simulink model "NBMS_App"  (R2026b)
settings: Solver=FixedStepDiscrete  StopTime=25  FixedStep=0.1
undefined symbols (not defined in the file): BMS_HVMosfet_STS_E, BMS_MODE_E, BMS_NM_Msg_E, Charger_Mode_Req_E
settings Model: ModifiedByFormat=Hari  Creator=hp  LastModifiedBy=Hari
settings OptimizationCC: DefaultParameterBehavior=Inlined  DifferentSizesBufferReuse=on  EfficientTunableParamExpr=on  EnhancedBackFolding=on  OptimizationCustomize=off  OptimizeBlockOrder=speed  PassReuseOutputArgsAs=Individual arguments  RemoveInternalMemoryZeroInit=on  RemoveRootLevelIOMemoryZeroInit=on
settings DebuggingCC: ParameterTunabilityLossMsg=error
settings SFSimCC: MATLABDynamicMemAlloc=off
settings RTWCC: Description=Embedded Coder  GenCodeOnly=on  PackageGeneratedCodeAndArtifacts=on  SystemTargetFile=ert.tlc  TemplateMakefile=ert_default_tmf
settings CodeAppCC: ForceParamTrailComments=on  IgnoreCustomStorageClasses=off  InsertBlockDesc=on  OperatorAnnotations=on  SFDataObjDesc=on  SimulinkDataObjDesc=on
settings ERTTargetCC: DynamicArrayContainerType=coder::array  GenerateSampleERTMain=on
settings ConfigComp: DVDefectChecker=on  DVDetectOutOfBounds=on  DVHarnessSource=Signal Editor  DVModelReferenceHarness=on  DVTestSuiteOptimization=Auto

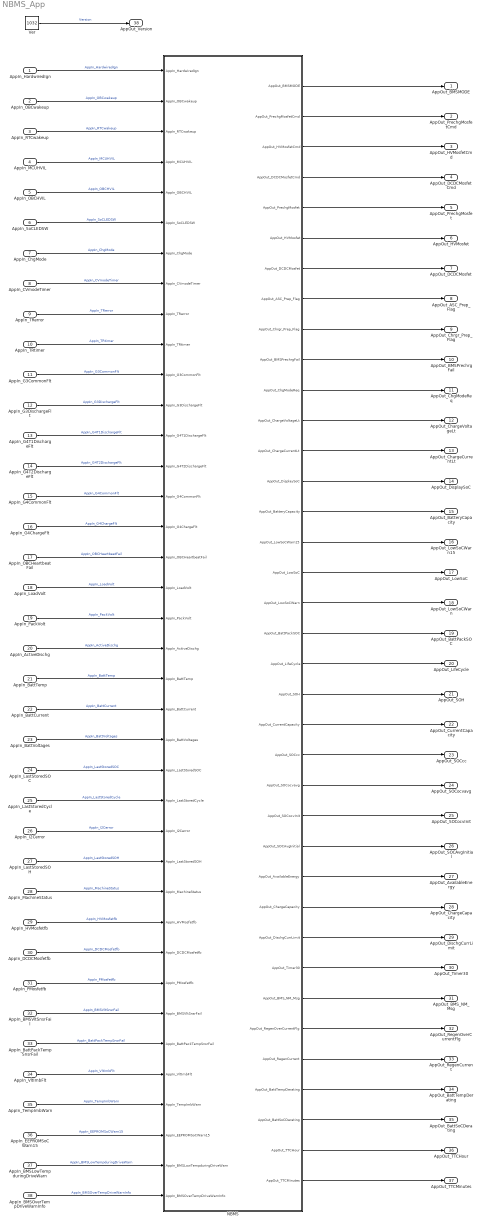
== system NBMS_App ==
  AppIn_HardwiredIgn : Inport  OutMin=0  OutMax=1  OutDataTypeStr=boolean
  AppIn_OBCwakeup : Inport  Port=2  OutDataTypeStr=Enum: OBC_E
  AppIn_RTCwakeup : Inport  Port=3  OutMin=0  OutMax=1  OutDataTypeStr=boolean
  AppIn_MCUHVIL : Inport  Port=4  OutMin=0  OutMax=1  OutDataTypeStr=boolean
  AppIn_OBCHVIL : Inport  Port=5  OutMin=0  OutMax=1  OutDataTypeStr=boolean
  AppIn_SoCLEDSW : Inport  Port=6  OutMin=0  OutMax=1  OutDataTypeStr=boolean
  AppIn_ChgMode : Inport  Port=7  OutDataTypeStr=Enum: Charger_Mode_E
  AppIn_CVmodeTimer : Inport  Port=8  OutDataTypeStr=Enum: CV_Mode_Timer_E
  AppIn_TRerror : Inport  Port=9  OutMin=0  OutMax=1  OutDataTypeStr=boolean
  AppIn_TRtimer : Inport  Port=10  OutMin=0  OutMax=1  OutDataTypeStr=boolean
  AppIn_G3CommonFlt : Inport  Port=11  OutMin=0  OutMax=1  OutDataTypeStr=boolean
  AppIn_G3DischargeFlt : Inport  Port=12  OutMin=0  OutMax=1  OutDataTypeStr=boolean
  AppIn_G4T1DischargeFlt : Inport  Port=13  OutMin=0  OutMax=1  OutDataTypeStr=boolean
  AppIn_G4T2DischargeFlt : Inport  Port=14  OutMin=0  OutMax=1  OutDataTypeStr=boolean
  AppIn_G4CommonFlt : Inport  Port=15  OutMin=0  OutMax=1  OutDataTypeStr=boolean
  AppIn_G4ChargeFlt : Inport  Port=16  OutMin=0  OutMax=1  OutDataTypeStr=boolean
  AppIn_OBCHeartbeatFail : Inport  Port=17  OutMin=0  OutMax=1  OutDataTypeStr=boolean
  AppIn_LoadVolt : Inport  Port=18  OutDataTypeStr=double
  AppIn_PackVolt : Inport  Port=19  OutDataTypeStr=double
  AppIn_ActiveDischg : Inport  Port=20  OutDataTypeStr=Enum: Active_DisChrg_E
  AppIn_BattTemp : Inport  Port=21  OutDataTypeStr=double  PortDimensions=[6,1]
  AppIn_BattCurrent : Inport  Port=22  OutDataTypeStr=double
  AppIn_BattVoltages : Inport  Port=23  OutDataTypeStr=double  PortDimensions=[20,1]
  AppIn_LastStoredSOC : Inport  Port=24  OutMin=0  OutMax=100  OutDataTypeStr=double
  AppIn_LastStoredCycle : Inport  Port=25  OutDataTypeStr=double
  AppIn_I2Cerror : Inport  Port=26  OutMin=0  OutMax=1  OutDataTypeStr=boolean
  AppIn_LastStoredSOH : Inport  Port=27  OutMin=0  OutMax=100  OutDataTypeStr=double
  AppIn_MachineStatus : Inport  Port=28  OutDataTypeStr=Enum: VDU_MACHINE_STS_E
  AppIn_HVMosfetfb : Inport  Port=29  OutMin=0  OutMax=1  OutDataTypeStr=boolean
  AppIn_DCDCMosfetfb : Inport  Port=30  OutMin=0  OutMax=1  OutDataTypeStr=boolean
  AppIn_PMosfetfb : Inport  Port=31  OutMin=0  OutMax=1  OutDataTypeStr=boolean
  AppIn_BMSVltSnsrFail : Inport  Port=32  OutMin=0  OutMax=1  OutDataTypeStr=boolean
  AppIn_BattPackTempSnsrFail : Inport  Port=33  OutMin=0  OutMax=1  OutDataTypeStr=boolean
  AppIn_VltImbFlt : Inport  Port=34  OutMin=0  OutMax=1  OutDataTypeStr=boolean
  AppIn_TempImbWarn : Inport  Port=35  OutMin=0  OutMax=1  OutDataTypeStr=boolean
  AppIn_EEPROMSoCWarn15 : Inport  Port=36  OutDataTypeStr=boolean
  AppIn_BMSLowTempduringDriveWarn : Inport  Port=37  OutDataTypeStr=boolean
  AppIn_BMSOverTempDriveWarnInfo : Inport  Port=38  OutDataTypeStr=boolean
  NBMS : Subsystem
  Ver : Constant  Value=1032
  AppOut_BMSMODE : Outport  SignalName=AppOut_BMSMODE  OutDataTypeStr=Enum: BMS_MODE_E
  AppOut_PrechgMosfetCmd : Outport  Port=2  SignalName=AppOut_PrechgMosfetCmd  OutMin=0  OutMax=1  OutDataTypeStr=boolean
  AppOut_HVMosfetCmd : Outport  Port=3  SignalName=AppOut_HVMosfetCmd  OutMin=0  OutMax=1  OutDataTypeStr=boolean
  AppOut_DCDCMosfetCmd : Outport  Port=4  SignalName=AppOut_DCDCMosfetCmd  OutMin=0  OutMax=1  OutDataTypeStr=boolean
  AppOut_PrechgMosfet : Outport  Port=5  SignalName=AppOut_PrechgMosfet  OutDataTypeStr=Enum: BMS_PMosfet_STS_E
  AppOut_HVMosfet : Outport  Port=6  SignalName=AppOut_HVMosfet  OutDataTypeStr=Enum: BMS_HVMosfet_STS_E
  AppOut_DCDCMosfet : Outport  Port=7  SignalName=AppOut_DCDCMosfet  OutDataTypeStr=Enum: BMS_DCDCMosfet_STS_E
  AppOut_ASC_Prep_Flag : Outport  Port=8  SignalName=AppOut_ASC_Prep_Flag  OutMin=0  OutMax=1  OutDataTypeStr=boolean
  AppOut_Chrgr_Prep_Flag : Outport  Port=9  SignalName=AppOut_Chrgr_Prep_Flag  OutMin=0  OutMax=1  OutDataTypeStr=boolean
  AppOut_BMSPrechrgFail : Outport  Port=10  SignalName=AppOut_BMSPrechrgFail  OutMin=0  OutMax=1  OutDataTypeStr=boolean
  AppOut_ChgModeReq : Outport  Port=11  SignalName=AppOut_ChgModeReq  OutDataTypeStr=Enum: Charger_Mode_Req_E
  AppOut_ChargeVoltageLt : Outport  Port=12  SignalName=AppOut_ChargeVoltageLt  OutDataTypeStr=double
  AppOut_ChargeCurrentLt : Outport  Port=13  SignalName=AppOut_ChargeCurrentLt  OutDataTypeStr=double
  AppOut_DisplaySoC : Outport  Port=14  SignalName=AppOut_DisplaySoC  OutMin=0  OutMax=100
  AppOut_BatteryCapacity : Outport  Port=15  SignalName=AppOut_BatteryCapacity
  AppOut_LowSoCWarn15 : Outport  Port=16  SignalName=AppOut_LowSoCWarn15  OutMin=0  OutMax=1  OutDataTypeStr=boolean
  AppOut_LowSoC : Outport  Port=17  SignalName=AppOut_LowSoC  OutMin=0  OutMax=1  OutDataTypeStr=boolean
  AppOut_LowSoCWarn : Outport  Port=18  SignalName=AppOut_LowSoCWarn  OutMin=0  OutMax=1  OutDataTypeStr=boolean
  AppOut_BattPackSOC : Outport  Port=19  SignalName=AppOut_BattPackSOC
  AppOut_LifeCycle : Outport  Port=20  SignalName=AppOut_LifeCycle
  AppOut_SOH : Outport  Port=21  SignalName=AppOut_SOH  OutMin=0  OutMax=100
  AppOut_CurrentCapacity : Outport  Port=22  SignalName=AppOut_CurrentCapacity  OutDataTypeStr=double
  AppOut_SOCcc : Outport  Port=23  SignalName=AppOut_SOCcc  OutDataTypeStr=fixdt(0,16,0.01,0)
  AppOut_SOCocvavg : Outport  Port=24  SignalName=AppOut_SOCocvavg  OutDataTypeStr=fixdt(0,16,0.01,0)
  AppOut_SOCocvInit : Outport  Port=25  SignalName=AppOut_SOCocvInit  OutDataTypeStr=double
  AppOut_SOCAvgInitial : Outport  Port=26  SignalName=AppOut_SOCAvgInitial  OutDataTypeStr=double
  AppOut_AvailableEnergy : Outport  Port=27  SignalName=AppOut_AvailableEnergy  OutDataTypeStr=double
  AppOut_ChargeCapacity : Outport  Port=28  SignalName=AppOut_ChargeCapacity  OutDataTypeStr=double
  AppOut_DischgCurrLimit : Outport  Port=29  SignalName=AppOut_DischgCurrLimit  OutDataTypeStr=double
  AppOut_Timer30 : Outport  Port=30  SignalName=AppOut_Timer30  OutDataTypeStr=double
  AppOut_BMS_NM_Msg : Outport  Port=31  SignalName=AppOut_BMS_NM_Msg  OutDataTypeStr=Enum: BMS_NM_Msg_E
  AppOut_RegenOverCurrentFlg : Outport  Port=32  SignalName=AppOut_RegenOverCurrentFlg  OutDataTypeStr=boolean
  AppOut_RegenCurrent : Outport  Port=33  SignalName=AppOut_RegenCurrent  OutDataTypeStr=double
  AppOut_BattTempDerating : Outport  Port=34  SignalName=AppOut_BattTempDerating  OutDataTypeStr=Enum: BMS_BattTempDerate_E
  AppOut_BattSoCDerating : Outport  Port=35  SignalName=AppOut_BattSoCDerating  OutDataTypeStr=Enum: BMS_BattSoCDerate_E
  AppOut_TTCHour : Outport  Port=36  SignalName=AppOut_TTCHour  OutDataTypeStr=double
  AppOut_TTCMinutes : Outport  Port=37  SignalName=AppOut_TTCMinutes  OutDataTypeStr=double
  AppOut_Version : Outport  Port=38  SignalName=AppOut_Version
  wires:
  AppIn_HardwiredIgn/1 -> NBMS/1(AppIn_HardwiredIgn)  "AppIn_HardwiredIgn"
  AppIn_OBCwakeup/1 -> NBMS/2(AppIn_OBCwakeup)  "AppIn_OBCwakeup"
  AppIn_OBCHeartbeatFail/1 -> NBMS/17(AppIn_OBCHeartbeatFail)  "AppIn_OBCHeartbeatFail"
  AppIn_G4ChargeFlt/1 -> NBMS/16(AppIn_G4ChargeFlt)  "AppIn_G4ChargeFlt"
  AppIn_G4T2DischargeFlt/1 -> NBMS/14(AppIn_G4T2DischargeFlt)  "AppIn_G4T2DischargeFlt"
  AppIn_G4CommonFlt/1 -> NBMS/15(AppIn_G4CommonFlt)  "AppIn_G4CommonFlt"
  AppIn_G3CommonFlt/1 -> NBMS/11(AppIn_G3CommonFlt)  "AppIn_G3CommonFlt"
  AppIn_G3DischargeFlt/1 -> NBMS/12(AppIn_G3DischargeFlt)  "AppIn_G3DischargeFlt"
  AppIn_TRtimer/1 -> NBMS/10(AppIn_TRtimer)  "AppIn_TRtimer"
  AppIn_TRerror/1 -> NBMS/9(AppIn_TRerror)  "AppIn_TRerror"
  AppIn_CVmodeTimer/1 -> NBMS/8(AppIn_CVmodeTimer)  "AppIn_CVmodeTimer"
  AppIn_ChgMode/1 -> NBMS/7(AppIn_ChgMode)  "AppIn_ChgMode"
  AppIn_SoCLEDSW/1 -> NBMS/6(AppIn_SoCLEDSW)  "AppIn_SoCLEDSW"
  AppIn_OBCHVIL/1 -> NBMS/5(AppIn_OBCHVIL)  "AppIn_OBCHVIL"
  AppIn_MCUHVIL/1 -> NBMS/4(AppIn_MCUHVIL)  "AppIn_MCUHVIL"
  AppIn_RTCwakeup/1 -> NBMS/3(AppIn_RTCwakeup)  "AppIn_RTCwakeup"
  AppIn_LoadVolt/1 -> NBMS/18(AppIn_LoadVolt)  "AppIn_LoadVolt"
  AppIn_PackVolt/1 -> NBMS/19(AppIn_PackVolt)  "AppIn_PackVolt"
  AppIn_ActiveDischg/1 -> NBMS/20(AppIn_ActiveDischg)  "AppIn_ActiveDischg"
  AppIn_BattTemp/1 -> NBMS/21(AppIn_BattTemp)  "AppIn_BattTemp"
  AppIn_LastStoredSOC/1 -> NBMS/24(AppIn_LastStoredSOC)  "AppIn_LastStoredSOC"
  AppIn_LastStoredCycle/1 -> NBMS/25(AppIn_LastStoredCycle)  "AppIn_LastStoredCycle"
  AppIn_I2Cerror/1 -> NBMS/26(AppIn_I2Cerror)  "AppIn_I2Cerror"
  AppIn_LastStoredSOH/1 -> NBMS/27(AppIn_LastStoredSOH)  "AppIn_LastStoredSOH"
  AppIn_MachineStatus/1 -> NBMS/28(AppIn_MachineStatus)  "AppIn_MachineStatus"
  AppIn_BattCurrent/1 -> NBMS/22(AppIn_BattCurrent)  "AppIn_BattCurrent"
  AppIn_BattVoltages/1 -> NBMS/23(AppIn_BattVoltages)  "AppIn_BattVoltages"
  NBMS/1(AppOut_BMSMODE) -> AppOut_BMSMODE/1
  NBMS/2(AppOut_PrechgMosfetCmd) -> AppOut_PrechgMosfetCmd/1
  NBMS/3(AppOut_HVMosfetCmd) -> AppOut_HVMosfetCmd/1
  NBMS/4(AppOut_DCDCMosfetCmd) -> AppOut_DCDCMosfetCmd/1
  NBMS/5(AppOut_PrechgMosfet) -> AppOut_PrechgMosfet/1
  NBMS/6(AppOut_HVMosfet) -> AppOut_HVMosfet/1
  NBMS/7(AppOut_DCDCMosfet) -> AppOut_DCDCMosfet/1
  NBMS/11(AppOut_ChgModeReq) -> AppOut_ChgModeReq/1
  NBMS/12(AppOut_ChargeVoltageLt) -> AppOut_ChargeVoltageLt/1
  NBMS/13(AppOut_ChargeCurrentLt) -> AppOut_ChargeCurrentLt/1
  NBMS/14(AppOut_DisplaySoC) -> AppOut_DisplaySoC/1
  NBMS/15(AppOut_BatteryCapacity) -> AppOut_BatteryCapacity/1
  NBMS/16(AppOut_LowSoCWarn15) -> AppOut_LowSoCWarn15/1
  NBMS/17(AppOut_LowSoC) -> AppOut_LowSoC/1
  NBMS/18(AppOut_LowSoCWarn) -> AppOut_LowSoCWarn/1
  NBMS/19(AppOut_BattPackSOC) -> AppOut_BattPackSOC/1
  NBMS/20(AppOut_LifeCycle) -> AppOut_LifeCycle/1
  NBMS/21(AppOut_SOH) -> AppOut_SOH/1
  NBMS/22(AppOut_CurrentCapacity) -> AppOut_CurrentCapacity/1
  NBMS/23(AppOut_SOCcc) -> AppOut_SOCcc/1
  NBMS/24(AppOut_SOCocvavg) -> AppOut_SOCocvavg/1
  NBMS/25(AppOut_SOCocvInit) -> AppOut_SOCocvInit/1
  NBMS/26(AppOut_SOCAvgInitial) -> AppOut_SOCAvgInitial/1
  NBMS/27(AppOut_AvailableEnergy) -> AppOut_AvailableEnergy/1
  NBMS/28(AppOut_ChargeCapacity) -> AppOut_ChargeCapacity/1
  NBMS/29(AppOut_DischgCurrLimit) -> AppOut_DischgCurrLimit/1
  NBMS/30(AppOut_Timer30) -> AppOut_Timer30/1
  AppIn_HVMosfetfb/1 -> NBMS/29(AppIn_HVMosfetfb)  "AppIn_HVMosfetfb"
  AppIn_DCDCMosfetfb/1 -> NBMS/30(AppIn_DCDCMosfetfb)  "AppIn_DCDCMosfetfb"
  AppIn_PMosfetfb/1 -> NBMS/31(AppIn_PMosfetfb)  "AppIn_PMosfetfb"
  NBMS/31(AppOut_BMS_NM_Msg) -> AppOut_BMS_NM_Msg/1
  NBMS/8(AppOut_ASC_Prep_Flag) -> AppOut_ASC_Prep_Flag/1
  NBMS/32(AppOut_RegenOverCurrentFlg) -> AppOut_RegenOverCurrentFlg/1
  NBMS/33(AppOut_RegenCurrent) -> AppOut_RegenCurrent/1
  AppIn_G4T1DischargeFlt/1 -> NBMS/13(AppIn_G4T1DischargeFlt)  "AppIn_G4T1DischargeFlt"
  NBMS/9(AppOut_Chrgr_Prep_Flag) -> AppOut_Chrgr_Prep_Flag/1
  AppIn_BMSVltSnsrFail/1 -> NBMS/32(AppIn_BMSVltSnsrFail)  "AppIn_BMSVltSnsrFail"
  AppIn_BattPackTempSnsrFail/1 -> NBMS/33(AppIn_BattPackTempSnsrFail)  "AppIn_BattPackTempSnsrFail"
  AppIn_VltImbFlt/1 -> NBMS/34(AppIn_VltImbFlt)  "AppIn_VltImbFlt"
  AppIn_TempImbWarn/1 -> NBMS/35(AppIn_TempImbWarn)  "AppIn_TempImbWarn"
  NBMS/10(AppOut_BMSPrechrgFail) -> AppOut_BMSPrechrgFail/1
  NBMS/34(AppOut_BattTempDerating) -> AppOut_BattTempDerating/1
  NBMS/35(AppOut_BattSoCDerating) -> AppOut_BattSoCDerating/1
  AppIn_EEPROMSoCWarn15/1 -> NBMS/36(AppIn_EEPROMSoCWarn15)  "AppIn_EEPROMSoCWarn15"
  AppIn_BMSLowTempduringDriveWarn/1 -> NBMS/37(AppIn_BMSLowTempduringDriveWarn)  "AppIn_BMSLowTempduringDriveWarn"
  AppIn_BMSOverTempDriveWarnInfo/1 -> NBMS/38(AppIn_BMSOverTempDriveWarnInfo)  "AppIn_BMSOverTempDriveWarnInfo"
  NBMS/36(AppOut_TTCHour) -> AppOut_TTCHour/1
  NBMS/37(AppOut_TTCMinutes) -> AppOut_TTCMinutes/1
  Ver/1 -> AppOut_Version/1  "Version"

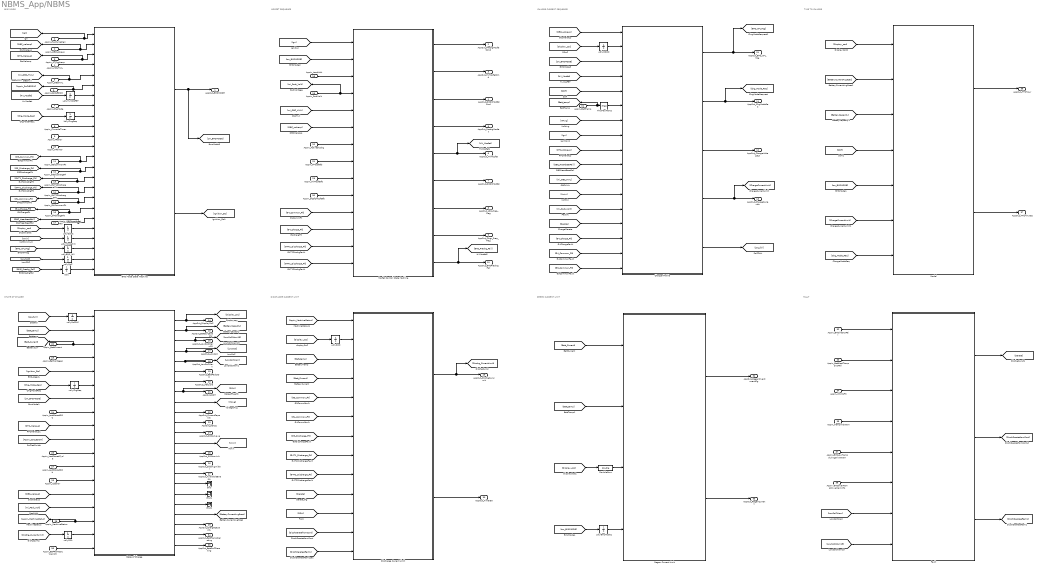
== system NBMS_App/NBMS ==
  note: STATE OF CHARGE
  note: CHARGE CURRENT SEQUENCE
  note: MOSFET SEQUENCE
  note: BMS MODE
  note: DISCHARGE CURRENT LIMIT
  note: REGEN CURRENT LIMIT
  note: FAULT
  note: TIME TO CHARGE
  AppIn_HardwiredIgn : Inport  OutDataTypeStr=boolean
  AppIn_OBCwakeup : Inport  Port=2  OutDataTypeStr=Enum: OBC_E
  AppIn_RTCwakeup : Inport  Port=3  OutDataTypeStr=boolean
  AppIn_MCUHVIL : Inport  Port=4  OutDataTypeStr=boolean
  AppIn_OBCHVIL : Inport  Port=5  OutDataTypeStr=boolean
  AppIn_SoCLEDSW : Inport  Port=6  OutDataTypeStr=boolean
  AppIn_ChgMode : Inport  Port=7  OutDataTypeStr=Enum: Charger_Mode_E
  AppIn_CVmodeTimer : Inport  Port=8  OutDataTypeStr=Enum: CV_Mode_Timer_E
  AppIn_TRerror : Inport  Port=9  OutDataTypeStr=boolean
  AppIn_TRtimer : Inport  Port=10  OutDataTypeStr=boolean
  AppIn_G3CommonFlt : Inport  Port=11  OutDataTypeStr=boolean
  AppIn_G3DischargeFlt : Inport  Port=12  OutDataTypeStr=boolean
  AppIn_G4T1DischargeFlt : Inport  Port=13
  AppIn_G4T2DischargeFlt : Inport  Port=14  OutDataTypeStr=boolean
  AppIn_G4CommonFlt : Inport  Port=15  OutDataTypeStr=boolean
  AppIn_G4ChargeFlt : Inport  Port=16  OutDataTypeStr=boolean
  AppIn_OBCHeartbeatFail : Inport  Port=17  OutDataTypeStr=boolean
  AppIn_LoadVolt : Inport  Port=18  OutDataTypeStr=double
  AppIn_PackVolt : Inport  Port=19  OutDataTypeStr=double
  AppIn_ActiveDischg : Inport  Port=20  OutDataTypeStr=Enum: Active_DisChrg_E
  AppIn_BattTemp : Inport  Port=21  OutDataTypeStr=double  PortDimensions=[6,1]
  AppIn_BattCurrent : Inport  Port=22  OutDataTypeStr=double
  AppIn_BattVoltages : Inport  Port=23  OutDataTypeStr=double  PortDimensions=[20,1]
  AppIn_LastStoredSOC : Inport  Port=24  OutDataTypeStr=double
  AppIn_LastStoredCycle : Inport  Port=25  OutDataTypeStr=double
  AppIn_I2Cerror : Inport  Port=26  OutDataTypeStr=boolean
  AppIn_LastStoredSOH : Inport  Port=27  OutDataTypeStr=double
  AppIn_MachineStatus : Inport  Port=28  OutDataTypeStr=Enum: VDU_MACHINE_STS_E
  AppIn_HVMosfetfb : Inport  Port=29  OutDataTypeStr=boolean
  AppIn_DCDCMosfetfb : Inport  Port=30  OutDataTypeStr=boolean
  AppIn_PMosfetfb : Inport  Port=31  OutDataTypeStr=boolean
  AppIn_BMSVltSnsrFail : Inport  Port=32  OutDataTypeStr=boolean
  AppIn_BattPackTempSnsrFail : Inport  Port=33  OutDataTypeStr=boolean
  AppIn_VltImbFlt : Inport  Port=34  OutDataTypeStr=boolean
  AppIn_TempImbWarn : Inport  Port=35  OutDataTypeStr=boolean
  AppIn_EEPROMSoCWarn15 : Inport  Port=36  OutDataTypeStr=boolean
  AppIn_BMSLowTempduringDriveWarn : Inport  Port=37  OutDataTypeStr=boolean
  AppIn_BMSOverTempDriveWarnInfo : Inport  Port=38  OutDataTypeStr=boolean
  BMS Mode State Machine : ModelReference  ModelNameDialog=NBMS_SM.slx  SimulationMode=Normal  ModelReferenceVersion=7.30
      settings: PortSchema="{\"entries\":[{\"content\":{\"sides\":[{\"content\":{\"connectorIds\":[\"In1\",\"In3\",\"In5\",\"In4\",\"In2\",\"In6\",\"In7\",\"In8\",\"In9\",\"In10\",\"In11\",\"In12\",\"In14\",\"In13\",\"In20\",\"In21\",\"In15\",\"In16\",\"In17\",\"In18\",\"In19\",\"In22\",\"In23\",\"In24\"]},\"type\":\"ConnectorPlacement.EquallySpacedRectSide\",\"uuid\":\"ecc493df-d9fb-4d48-bfac-df3b040d40be\"},{\"content\":{\"connectorIds\":[\"Out1\",\"Out2\"],\"side\":\"RIGHT\"},\"type\":\"ConnectorPlacement.EquallySpacedRectSide\",\"uuid\":\"d66811ed-6c1c-40f3-961a-d24c32966bca\"},{\"content\":{\"side\":\"TOP\"},\"type\":\"ConnectorPlacement.EquallySpacedRectSide\",\"uuid\":\"c4a8e5f3-9cec-48fd-8595-92a124cd4df9\"}]},\"type\":\"ConnectorPlacement.EquallySpacedConnector\",\"uuid\":\"a32d3843-be82-4c44-a288-33a33938b272\"}],\"packageUris\":[\"http://schema.mathworks.com/mf0/Connector/R2020b\"],\"version\":\"1.0\"}"
  Charger Profile : ModelReference  ModelNameDialog=NBMS_CCCV.slx  SimulationMode=Normal  ModelReferenceVersion=7.36
      settings: PortSchema="{\"entries\":[{\"content\":{\"sides\":[{\"content\":{\"connectorIds\":[\"In1\",\"In2\",\"In3\",\"In4\",\"In5\",\"In6\",\"In7\",\"In8\",\"In9\",\"In10\",\"In11\",\"In12\",\"In13\",\"In14\",\"In15\",\"In16\",\"In17\"]},\"type\":\"ConnectorPlacement.EquallySpacedRectSide\",\"uuid\":\"373b2497-420a-45a3-ad28-05a6ac9a8d10\"},{\"content\":{\"connectorIds\":[\"Out1\",\"Out2\",\"Out3\",\"Out5\",\"Out4\"],\"side\":\"RIGHT\"},\"type\":\"ConnectorPlacement.EquallySpacedRectSide\",\"uuid\":\"9fe77b2b-0f95-4ff2-ba28-d6de646e2ea4\"},{\"content\":{\"side\":\"TOP\"},\"type\":\"ConnectorPlacement.EquallySpacedRectSide\",\"uuid\":\"8ddc6517-5312-4b06-8c0f-7070160c61ca\"}]},\"type\":\"ConnectorPlacement.EquallySpacedConnector\",\"uuid\":\"1c52dcf7-dcaa-4bbc-ab99-189758e4b109\"}],\"packageUris\":[\"http://schema.mathworks.com/mf0/Connector/R2020b\"],\"version\":\"1.0\"}"
  Discharge Current Limit : ModelReference  ModelNameDialog=NBMS_DCL.slx  SimulationMode=Normal  ModelReferenceVersion=7.26
  DoubleConv : DataTypeConversion  OutDataTypeStr=double  SaturateOnIntegerOverflow=off  RndMeth=Floor
  Fault : ModelReference  ModelNameDialog=NBMS_Fault.slx  SimulationMode=Normal  ModelReferenceVersion=1.6
  FindMaxTemp : MinMax  Function=max
  Gnd : Terminator
  Gnd1 : Terminator
  Gnd2 : Terminator
  Model : ModelReference  ModelNameDialog=NBMS_TTC.slx  SimulationMode=Normal  ModelReferenceVersion=1.10
  Mosfet Control State Machine : ModelReference  ModelNameDialog=NBMS_MosfetSeq.slx  SimulationMode=Normal  ModelReferenceVersion=7.47
  Regen Current Limit : ModelReference  ModelNameDialog=NBMS_Regen.slx  SimulationMode=Normal  ModelReferenceVersion=7.14
  State of Charge : ModelReference  ModelNameDialog=NBMS_SoC.slx  SimulationMode=Normal  ModelReferenceVersion=7.110
      settings: PortSchema="{\"entries\":[{\"content\":{\"sides\":[{\"content\":{\"connectorIds\":[\"In1\",\"In2\",\"In3\",\"In4\",\"In5\",\"In6\",\"In7\",\"In8\",\"In16\",\"In17\",\"In9\",\"In11\",\"In10\",\"In12\",\"In13\",\"In14\",\"In15\",\"In18\"]},\"type\":\"ConnectorPlacement.EquallySpacedRectSide\",\"uuid\":\"295ac103-dd5b-4923-8c3d-4e88aeddbae6\"},{\"content\":{\"connectorIds\":[\"Out1\",\"Out2\",\"Out3\",\"Out4\",\"Out5\",\"Out6\",\"Out7\",\"Out8\",\"Out9\",\"Out10\",\"Out11\",\"Out12\",\"Out13\",\"Out14\",\"Out15\",\"Out16\",\"Out17\",\"Out18\",\"Out19\",\"Out20\",\"Out21\",\"Out22\",\"Out23\"],\"side\":\"RIGHT\"},\"type\":\"ConnectorPlacement.EquallySpacedRectSide\",\"uuid\":\"285b0d34-fee8-4213-b554-c61a8df57e9d\"},{\"content\":{\"side\":\"TOP\"},\"type\":\"ConnectorPlacement.EquallySpacedRectSide\",\"uuid\":\"eafcffe6-a650-4781-a196-43539fe9012d\"}]},\"type\":\"ConnectorPlacement.EquallySpacedConnector\",\"uuid\":\"1d9f679a-0ec3-4923-807e-88f567b97b85\"}],\"packageUris\":[\"http://schema.mathworks.com/mf0/Connector/R2020b\"],\"version\":\"1.0\"}"
  Udly : UnitDelay  SampleTime=-1
  UdlyChrgReq : UnitDelay  InitialCondition=Charger_Mode_Req_E.Disabled  SampleTime=-1
  uDlyDSOC : UnitDelay  SampleTime=-1
  udlyBMS_NM : UnitDelay  InitialCondition=BMS_NM_Msg_E.SLEEP  SampleTime=-1
  udlyBmsMode1 : UnitDelay  InitialCondition=BMS_MODE_E.BMS_SLEEP  SampleTime=-1
  udlyChgReq : UnitDelay  InitialCondition=Charger_Mode_Req_E.Disabled  SampleTime=-1
  udlyDCL : UnitDelay  SampleTime=-1
  udlyDSoC : UnitDelay  SampleTime=-1
  udlyHvMOSFET : UnitDelay  InitialCondition=BMS_HVMosfet_STS_E.HV_DISCONNECTED  SampleTime=-1
  udlyMinCellVt : UnitDelay  SampleTime=-1
  udlySOC : UnitDelay  SampleTime=-1
  udlySoC : UnitDelay  SampleTime=-1
  udlySoCFull : UnitDelay  SampleTime=-1
  AppOut_BMSMODE : Outport  OutDataTypeStr=Enum: BMS_MODE_E
  AppOut_PrechgMosfetCmd : Outport  Port=2  OutDataTypeStr=boolean
  AppOut_HVMosfetCmd : Outport  Port=3  OutDataTypeStr=boolean
  AppOut_DCDCMosfetCmd : Outport  Port=4  OutDataTypeStr=boolean
  AppOut_PrechgMosfet : Outport  Port=5  OutDataTypeStr=Enum: BMS_PMosfet_STS_E
  AppOut_HVMosfet : Outport  Port=6  OutDataTypeStr=Enum: BMS_HVMosfet_STS_E
  AppOut_DCDCMosfet : Outport  Port=7  OutDataTypeStr=Enum: BMS_DCDCMosfet_STS_E
  AppOut_ASC_Prep_Flag : Outport  Port=8  OutDataTypeStr=boolean
  AppOut_Chrgr_Prep_Flag : Outport  Port=9
  AppOut_BMSPrechrgFail : Outport  Port=10  OutDataTypeStr=boolean
  AppOut_ChgModeReq : Outport  Port=11  OutDataTypeStr=Enum: Charger_Mode_Req_E
  AppOut_ChargeVoltageLt : Outport  Port=12  OutDataTypeStr=double
  AppOut_ChargeCurrentLt : Outport  Port=13  OutDataTypeStr=double
  AppOut_DisplaySoC : Outport  Port=14
  AppOut_BatteryCapacity : Outport  Port=15
  AppOut_LowSoCWarn15 : Outport  Port=16  OutDataTypeStr=boolean
  AppOut_LowSoC : Outport  Port=17  OutDataTypeStr=boolean
  AppOut_LowSoCWarn : Outport  Port=18  OutDataTypeStr=boolean
  AppOut_BattPackSOC : Outport  Port=19
  AppOut_LifeCycle : Outport  Port=20
  AppOut_SOH : Outport  Port=21
  AppOut_CurrentCapacity : Outport  Port=22  OutDataTypeStr=double
  AppOut_SOCcc : Outport  Port=23  OutDataTypeStr=fixdt(0,16,0.01,0)
  AppOut_SOCocvavg : Outport  Port=24  OutDataTypeStr=fixdt(0,16,0.01,0)
  AppOut_SOCocvInit : Outport  Port=25  OutDataTypeStr=double
  AppOut_SOCAvgInitial : Outport  Port=26  OutDataTypeStr=double
  AppOut_AvailableEnergy : Outport  Port=27  OutDataTypeStr=double
  AppOut_ChargeCapacity : Outport  Port=28  OutDataTypeStr=double
  AppOut_DischgCurrLimit : Outport  Port=29  OutDataTypeStr=double
  AppOut_Timer30 : Outport  Port=30  OutDataTypeStr=double
  AppOut_BMS_NM_Msg : Outport  Port=31  OutDataTypeStr=Enum: BMS_NM_Msg_E
  AppOut_RegenOverCurrentFlg : Outport  Port=32  OutDataTypeStr=boolean
  AppOut_RegenCurrent : Outport  Port=33  OutDataTypeStr=double
  AppOut_BattTempDerating : Outport  Port=34  OutDataTypeStr=Enum: BMS_BattTempDerate_E
  AppOut_BattSoCDerating : Outport  Port=35  OutDataTypeStr=Enum: BMS_BattSoCDerate_E
  AppOut_TTCHour : Outport  Port=36  OutDataTypeStr=double
  AppOut_TTCMinutes : Outport  Port=37  OutDataTypeStr=double
  wires:
  State of Charge/5 -> [LowSoCWarn], AppOut_LowSoCWarn/1
  State of Charge/11 -> AppOut_SOCcc/1
  State of Charge/16 -> AppOut_AvailableEnergy/1
  [VtAvg] -> Charger Profile/7
  State of Charge/13 -> [Vmin]
  State of Charge/4 -> [LowSoC], AppOut_LowSoC/1
  AppIn_BattVoltages/1 -> State of Charge/4
  AppIn_I2Cerror/1 -> State of Charge/10
  State of Charge/12 -> AppOut_SOCocvavg/1
  [Batt_temp] -> State of Charge/2
  [Chg_Mode_Req] -> udlyChgReq/1
  State of Charge/15 -> AppOut_SOCAvgInitial/1
  [soc_full] -> udlySoCFull/1
  State of Charge/1 -> [Display_soc], AppOut_DisplaySoC/1
  State of Charge/8 -> AppOut_SOH/1, [SOH]
  FindMaxTemp/1 -> Charger Profile/6  "MaxTemp"
  State of Charge/10 -> AppOut_CurrentCapacity/1
  State of Charge/2 -> [BatteryCapacity], AppOut_BatteryCapacity/1
  AppIn_LastStoredSOC/1 -> State of Charge/8
  State of Charge/21 -> AppOut_ChargeCapacity/1
  AppIn_BattCurrent/1 -> [Batt_Current], State of Charge/3
  Charger Profile/4 -> [soc_full]
  [Ignition_Sts] -> State of Charge/5
  AppIn_MachineStatus/1 -> State of Charge/14, [AppIn_MachineStatus]
  [mi_Pack_Volt] -> State of Charge/13
  AppIn_LastStoredCycle/1 -> State of Charge/9
  [OBC_wakeup] -> State of Charge/12
  State of Charge/17 -> Gnd/1
  [SOH] -> Charger Profile/5
  AppIn_BattTemp/1 -> [Batt_temp], FindMaxTemp/1
  State of Charge/7 -> AppOut_LifeCycle/1
  Charger Profile/2 -> [Chg_Mode_Req], AppOut_ChgModeReq/1
  [sm_BMSMODE] -> Charger Profile/3
  [Dischg_CurrentLimit] -> udlyDCL/1
  uDlyDSOC/1 -> Charger Profile/2  "DisplaySoC"
  [OBC_wakeup] -> Charger Profile/1
  [HV_Mosfet] -> Charger Profile/4
  AppIn_G4ChargeFlt/1 -> [G4_Charge_Flt], BMS Mode State Machine/16
  AppIn_OBCHVIL/1 -> [mi_OBC_HVIL], BMS Mode State Machine/2
  AppIn_OBCHeartbeatFail/1 -> [OBC_HeartbeatFail], BMS Mode State Machine/17
  AppIn_CVmodeTimer/1 -> BMS Mode State Machine/10
  AppIn_G3CommonFlt/1 -> [G3_Common_Flt], BMS Mode State Machine/14
  AppIn_G4CommonFlt/1 -> [G4_Common_Flt], BMS Mode State Machine/15
  AppIn_MCUHVIL/1 -> BMS Mode State Machine/4
  udlyDSoC/1 -> BMS Mode State Machine/18  "DisplaySoC"
  AppIn_HardwiredIgn/1 -> [Ign], BMS Mode State Machine/1
  AppIn_OBCwakeup/1 -> [OBC_wakeup], BMS Mode State Machine/3
  [Display_soc] -> uDlyDSOC/1
  [sm_BMSMODE] -> State of Charge/7  "PrevBmsMode"
  [Chg_Mode_Req] -> UdlyChrgReq/1
  State of Charge/20 -> [BatteryCurrentAvg5sec]
  State of Charge/9 -> [VtAvg]
  udlySoCFull/1 -> State of Charge/1  "PrevSoCFul"
  [mi_OBC_HVIL] -> Mosfet Control State Machine/5
  [Ign] -> Mosfet Control State Machine/1
  [OBC_wakeup] -> Mosfet Control State Machine/6
  Charger Profile/3 -> AppOut_ChargeVoltageLt/1
  State of Charge/6 -> AppOut_BattPackSOC/1
  Mosfet Control State Machine/2 -> AppOut_HVMosfetCmd/1
  State of Charge/19 -> Gnd2/1
  State of Charge/18 -> Gnd1/1
  Mosfet Control State Machine/1 -> AppOut_PrechgMosfetCmd/1
  AppIn_TRerror/1 -> BMS Mode State Machine/11
  State of Charge/14 -> AppOut_SOCocvInit/1
  [Display_soc] -> udlyDSoC/1
  [sm_BMSMODE] -> Mosfet Control State Machine/2  "BMSMode"
  AppIn_SoCLEDSW/1 -> BMS Mode State Machine/6, [AppIn_SoCLEDSW]
  AppIn_PackVolt/1 -> [mi_Pack_Volt], Mosfet Control State Machine/4
  Mosfet Control State Machine/5 -> AppOut_HVMosfet/1, [HV_Mosfet]
  Mosfet Control State Machine/4 -> AppOut_PrechgMosfet/1
  AppIn_ChgMode/1 -> BMS Mode State Machine/8
  Charger Profile/5 -> [ChargeCurrentLimit], AppOut_ChargeCurrentLt/1
  AppIn_G4T2DischargeFlt/1 -> BMS Mode State Machine/21, [G4T2_Discharge_Flt]
  State of Charge/3 -> [LowSoCWarn15], AppOut_LowSoCWarn15/1
  AppIn_LoadVolt/1 -> Mosfet Control State Machine/3
  udlyChgReq/1 -> State of Charge/6  "PrevChgReq"
  AppIn_RTCwakeup/1 -> [RTC_Wakeup], BMS Mode State Machine/5
  AppIn_TRtimer/1 -> BMS Mode State Machine/12
  Mosfet Control State Machine/6 -> AppOut_DCDCMosfet/1
  Mosfet Control State Machine/3 -> AppOut_DCDCMosfetCmd/1
  AppIn_ActiveDischg/1 -> Mosfet Control State Machine/7
  AppIn_G3DischargeFlt/1 -> BMS Mode State Machine/13, [G3_Discharge_Flt]
  BMS Mode State Machine/1 -> [sm_BMSMODE], AppOut_BMSMODE/1
  [HV_Mosfet] -> udlyHvMOSFET/1
  AppIn_LastStoredSOH/1 -> State of Charge/11
  [AppIn_MachineStatus] -> Discharge Current Limit/1
  [Display_soc] -> udlySOC/1
  [Batt_Current] -> Discharge Current Limit/4
  Discharge Current Limit/1 -> [Dischg_CurrentLimit], AppOut_DischgCurrLimit/1
  Discharge Current Limit/2 -> AppOut_Timer30/1
  [Batt_temp] -> Discharge Current Limit/3
  udlyDCL/1 -> State of Charge/15  "PrevDCL"
  udlySOC/1 -> Discharge Current Limit/2  "SoC"
  UdlyChrgReq/1 -> BMS Mode State Machine/9  "ChrgReq"
  AppIn_HVMosfetfb/1 -> Mosfet Control State Machine/9
  AppIn_DCDCMosfetfb/1 -> Mosfet Control State Machine/10
  AppIn_PMosfetfb/1 -> Mosfet Control State Machine/8
  Charger Profile/1 -> [BMS_NM_Msg], AppOut_BMS_NM_Msg/1
  [Ign] -> Charger Profile/8
  [mi_Pack_Volt] -> Charger Profile/13
  [mi_OBC_HVIL] -> Charger Profile/11
  [OBC_HeartbeatFail] -> Charger Profile/10
  [RTC_Wakeup] -> Charger Profile/9
  [Vmin] -> Charger Profile/12
  [Vmin] -> udlyMinCellVt/1
  Mosfet Control State Machine/7 -> AppOut_ASC_Prep_Flag/1
  [Batt_Current] -> Regen Current Limit/1
  [Batt_temp] -> Regen Current Limit/2
  [Display_soc] -> DoubleConv/1
  DoubleConv/1 -> Regen Current Limit/3  "SoC"
  [sm_BMSMODE] -> udlyBmsMode1/1
  udlyBmsMode1/1 -> Regen Current Limit/4  "PrevBmsMode"
  Regen Current Limit/1 -> AppOut_RegenOverCurrentFlg/1
  Regen Current Limit/2 -> AppOut_RegenCurrent/1
  AppIn_G4T1DischargeFlt/1 -> [G4T1_Discharge_Flt], BMS Mode State Machine/20
  [G4_Charge_Flt] -> Charger Profile/15
  [G4_Common_Flt] -> Charger Profile/16
  [G3_Common_Flt] -> Charger Profile/17
  [G4_Common_Flt] -> Mosfet Control State Machine/11
  [G4_Charge_Flt] -> Mosfet Control State Machine/12
  Mosfet Control State Machine/8 -> AppOut_Chrgr_Prep_Flag/1
  [G4T2_Discharge_Flt] -> Mosfet Control State Machine/13
  [G4T1_Discharge_Flt] -> Mosfet Control State Machine/14
  [G3_Common_Flt] -> Discharge Current Limit/5
  [G4_Common_Flt] -> Discharge Current Limit/6
  [G4T2_Discharge_Flt] -> Discharge Current Limit/9
  [G4T1_Discharge_Flt] -> Discharge Current Limit/8
  [G3_Discharge_Flt] -> Discharge Current Limit/7
  AppIn_BMSVltSnsrFail/1 -> Fault/1
  AppIn_BattPackTempSnsrFail/1 -> Fault/2
  AppIn_VltImbFlt/1 -> Fault/3
  AppIn_TempImbWarn/1 -> Fault/4
  Fault/1 -> [Derate]
  [Derate] -> Charger Profile/14
  Mosfet Control State Machine/9 -> [BMS_Prechg_Fail], AppOut_BMSPrechrgFail/1
  udlyHvMOSFET/1 -> BMS Mode State Machine/7  "HVMosfet"
  udlyMinCellVt/1 -> BMS Mode State Machine/19  "MinCellVt"
  BMS Mode State Machine/2 -> [Ignition_Sts]
  [Derate] -> Discharge Current Limit/10
  State of Charge/22 -> AppOut_BattTempDerating/1
  State of Charge/23 -> AppOut_BattSoCDerating/1
  [RTC_Wakeup] -> State of Charge/16
  [AppIn_SoCLEDSW] -> State of Charge/17
  [BMS_NM_Msg] -> udlyBMS_NM/1
  udlyBMS_NM/1 -> BMS Mode State Machine/22  "BMS_NM_Msg"
  AppIn_EEPROMSoCWarn15/1 -> State of Charge/18  "EEPROMSoCWarn15"
  [SOH] -> Discharge Current Limit/11
  Fault/2 -> [DischDeratefromCont]
  Fault/3 -> [DischDerateafterX1]
  AppIn_BMSLowTempduringDriveWarn/1 -> Fault/5
  [LowSoCWarn] -> Fault/7
  AppIn_BMSOverTempDriveWarnInfo/1 -> Fault/6
  [LowSoCWarn15] -> Fault/8
  [DischDeratefromCont] -> Discharge Current Limit/12
  [DischDerateafterX1] -> Discharge Current Limit/13
  [LowSoC] -> udlySoC/1
  udlySoC/1 -> BMS Mode State Machine/23
  [Display_soc] -> Model/1
  [BatteryCurrentAvg5sec] -> Model/2
  [BatteryCapacity] -> Model/3
  [SOH] -> Model/4
  [sm_BMSMODE] -> Model/5
  [ChargeCurrentLimit] -> Model/6
  [Chg_Mode_Req] -> Model/7
  Model/1 -> AppOut_TTCHour/1  "TTCHour"
  Model/2 -> AppOut_TTCMinutes/1  "TTCMinutes"
  [BMS_Prechg_Fail] -> Udly/1
  Udly/1 -> BMS Mode State Machine/24
